simulink model "Single_Phase_HERIC_Inverter"  (R2023b)
settings: Solver=VariableStepAuto  StartTime=0.0  StopTime=0.5  RelTol=1e-3
libraries: spsSeriesRLCBranchLib x5, spsVoltageMeasurementLib x4, spsCurrentMeasurementLib x2, spsIGBTDiodeLib x2, spsMeanLib x2, spsACVoltageSourceLib x1, spsDCVoltageSourceLib x1, spsUniversalBridgeLib x1, powerlib_extras x1, spsRMSLib x1, spsTHDLib x1, spspowerguiLib x1
settings Model: SimulationMode=accelerator  Creator=abc6820292  LastModifiedBy=Qu
settings DataIOCC: ReturnWorkspaceOutputs=off
settings DebuggingCC: UnconnectedInputMsg=warning  UnconnectedOutputMsg=warning  UnconnectedLineMsg=warning
settings ModelReferenceCC: EnableRefExpFcnMdlSchedulingChecks=on
settings RTWCC: DLArmComputeVersion=19.05

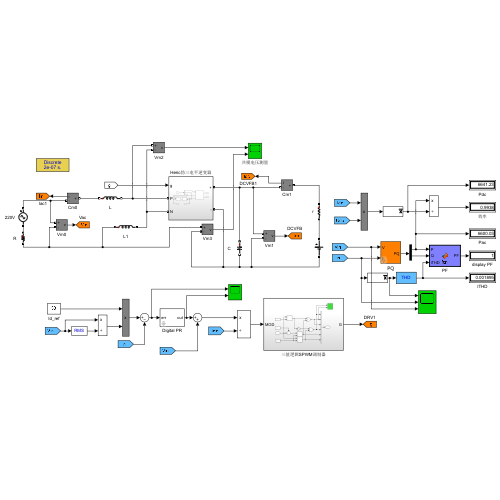
[thumbnail: Simulink's stored preview of the top-level diagram]
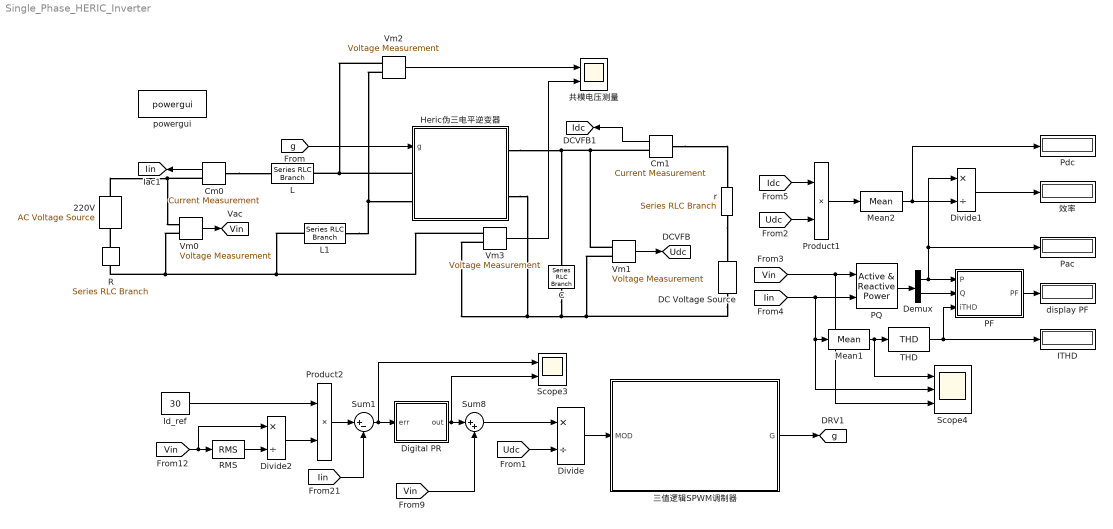
== system Single_Phase_HERIC_Inverter ==
  220V : spsACVoltageSourceLib/AC Voltage Source  Amplitude=220*1.414  Phase=0  Frequency=50  SampleTime=0  Measurements=None  BusType=swing  Pref=10e3  Qref=0  Qmin=-inf  Qmax=+inf
  C : spsSeriesRLCBranchLib/Series RLC Branch  LConnTagsString=__new0  RConnTagsString=__new0  BranchType=C  Resistance=0.01  Inductance=7e-4  SetiL0=off  InitialCurrent=0  Capacitance=2e-3  Setx0=on  InitialVoltage=360  Measurements=None
  Cm0 : spsCurrentMeasurementLib/Current Measurement  PhasorSimulation=off  OutputType=Complex  PSBequivalent=0
  Cm1 : spsCurrentMeasurementLib/Current Measurement  PhasorSimulation=off  OutputType=Complex  PSBequivalent=0
  DC Voltage Source : spsDCVoltageSourceLib/DC Voltage Source  Amplitude=360  Measurements=None
  Demux : Demux  Outputs=2
  Digital PR : Subsystem  mask{Kp=6, Kr=100, Wc=5, Ts=1/40000, Upper=400, Lower=-400}
      mask DialogControl ParameterGroupVar Prompt: 参数
  Divide : Product  Inputs=*/
  Divide1 : Product  Inputs=*/
  Divide2 : Product  Inputs=*/
  Heric伪三电平逆变器 : Subsystem
  ITHD : Display
  Id_ref : Constant  Value=30
  L : spsSeriesRLCBranchLib/Series RLC Branch  LConnTagsString=__new0  RConnTagsString=__new0  BranchType=L  Resistance=0.05  Inductance=3e-4  SetiL0=off  InitialCurrent=0  Capacitance=1e-3  Setx0=off  InitialVoltage=0  Measurements=None
  L1 : spsSeriesRLCBranchLib/Series RLC Branch  LConnTagsString=__new0  RConnTagsString=__new0  BranchType=L  Resistance=0.05  Inductance=3e-4  SetiL0=off  InitialCurrent=0  Capacitance=1e-3  Setx0=off  InitialVoltage=0  Measurements=None
  Mean1 : spsMeanLib/Mean  Freq=10000  Vinit=0  Ts=0
  Mean2 : spsMeanLib/Mean  Freq=50  Vinit=0  Ts=0
  PF : MATLAB Function  TreatAsAtomicUnit=on
  PQ : powerlib_extras/Measurements/Active & Reactive Power  f1=50
  Pac : Display
      settings: Format=bank
  Pdc : Display
      settings: Format=bank
  Product1 : Product  RndMeth=Zero
  Product2 : Product  RndMeth=Zero
  R : spsSeriesRLCBranchLib/Series RLC Branch  LConnTagsString=__new0  RConnTagsString=__new0  BranchType=R  Resistance=0.01  Inductance=7e-4  SetiL0=off  InitialCurrent=0  Capacitance=1e-8  Setx0=off  InitialVoltage=200  Measurements=None
  RMS : spsRMSLib/RMS  TrueRMS=off  Freq=50  RMSInit=220  Ts=0
  Scope3 : Scope  NumInputPorts=2
  Scope4 : Scope  NumInputPorts=3
  Sum1 : Sum  Inputs=|+-
  Sum8 : Sum  Inputs=|++
  THD : spsTHDLib/THD  Freq=50  Ts=0
  Vm{0..3} (4 alike) : spsVoltageMeasurementLib/Voltage Measurement  PhasorSimulation=off  OutputType=Complex  PSBequivalent=0
  display PF : Display
  powergui : spspowerguiLib/powergui  SimulationMode=Discrete  SampleTime=2e-7  frequency=60  Iterations=50  frequencyindice=0  Pbase=100e6  ErrMax=1e-4  UnitsV=kV  UnitsW=MW  buscounter=0  FunctionMessages=off  echomessages=off  EnableUseOfTLC=off  CurrentSourceSwitches=off  DisableSnubberDevices=off  DisableRonSwitches=off  DisableVfSwitches=off  DisplayEquations=off  AutomaticDiscreteSolvers=off  SolverType=Tustin/Backward Euler (TBE)  Interpol=off  ExternalGateDelay=off  methode=off  Ts=0  x0status=blocks  SPID=off  SwTol=0  HookPort=off  NonlinearTolerance=1e-4  nMaxIteration=100  ContinueOnMaxIteration=off  RestoreLinks=warning  ResistiveCurrentMeasurement=off  Frange=[0:2:500]  Ylog=off  Xlog=on  ShowGrid=off  save=off  variable=ZData  structure=QQQQQ  ZoomFFT=off  StartTime=0.5  cycles=15  DisplayStyle=1  fundamental=50  FreqAxis=off  MaxFrequency=1000  frequencyindicesteady=1  RmsSteady=1  display=off
  r : spsSeriesRLCBranchLib/Series RLC Branch  LConnTagsString=__new0  RConnTagsString=__new0  BranchType=R  Resistance=0.05  Inductance=1e-4  SetiL0=off  InitialCurrent=0  Capacitance=1e-3  Setx0=off  InitialVoltage=0  Measurements=None
  三值逻辑SPWM调制器 : Subsystem
  共模电压测量 : Scope  NumInputPorts=2
  效率 : Display
  tag scope: Idc=global, Iin=global, Udc=global, Vin=global, g=global
  wires:
  [g] -> Heric伪三电平逆变器/1(g)
  Vm0/1 -> [Vin]
  Demux/2 -> PF/2(Q)
  PF/1(PF) -> display PF/1
  PQ/1 -> Demux/1
  THD/1 -> ITHD/1, PF/3(iTHD)
  [Vin] -> Scope4/3, PQ/1
  Demux/1 -> Divide1/1, Pac/1, PF/1(P)
  Vm1/1 -> [Udc]
  三值逻辑SPWM调制器/1(G) -> [g]
  Cm0/1 -> [Iin]
  Divide/1 -> 三值逻辑SPWM调制器/1(MOD)
  [Udc] -> Divide/2
  [Iin] -> Sum1/2
  [Iin] -> Scope4/2, Mean1/1, PQ/2
  Sum8/1 -> Divide/1
  [Vin] -> Sum8/2
  [Vin] -> Divide2/1, RMS/1
  RMS/1 -> Divide2/2
  Divide2/1 -> Product2/2
  Id_ref/1 -> Product2/1
  Mean1/1 -> Scope4/1, THD/1
  Sum1/1 -> Digital PR/1(err), Scope3/1
  Product2/1 -> Sum1/1
  Vm2/1 -> 共模电压测量/1
  Vm3/1 -> 共模电压测量/2
  Digital PR/1(out) -> Scope3/2, Sum8/1
  Cm1/1 -> [Idc]
  [Udc] -> Product1/2
  [Idc] -> Product1/1
  Product1/1 -> Mean2/1
  Mean2/1 -> Pdc/1, Divide1/2
  Divide1/1 -> 效率/1
  connections:
  Vm1/LConn1 -- Heric伪三电平逆变器/RConn1 -- C/LConn1 -- Cm1/RConn1
  DC Voltage Source/LConn1 -- C/RConn1 -- Vm3/LConn2 -- Heric伪三电平逆变器/RConn2 -- Vm1/LConn2
  Cm0/RConn1 -- 220V/RConn1 -- Vm0/LConn1
  Vm2/LConn2 -- L1/RConn1 -- Heric伪三电平逆变器/LConn2
  Cm0/LConn1 -- L/LConn1
  r/RConn1 -- DC Voltage Source/RConn1
  L/RConn1 -- Heric伪三电平逆变器/LConn1 -- Vm2/LConn1
  R/LConn1 -- 220V/LConn1
  Vm0/LConn2 -- Vm3/LConn1 -- L1/LConn1 -- R/RConn1
  Cm1/LConn1 -- r/LConn1

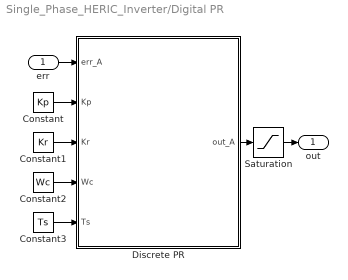
== system Single_Phase_HERIC_Inverter/Digital PR ==
  err : Inport
  Constant : Constant  Value=Kp
  Constant1 : Constant  Value=Kr
  Constant2 : Constant  Value=Wc
  Constant3 : Constant  Value=Ts
  Discrete PR : MATLAB Function  TreatAsAtomicUnit=on
  Saturation : Saturate  UpperLimit=Upper  LowerLimit=Lower
  out : Outport
  wires:
  Constant1/1 -> Discrete PR/3(Kr)
  Constant3/1 -> Discrete PR/5(Ts)
  Constant/1 -> Discrete PR/2(Kp)
  Constant2/1 -> Discrete PR/4(Wc)
  Discrete PR/1(out_A) -> Saturation/1
  Saturation/1 -> out/1
  err/1 -> Discrete PR/1(err_A)

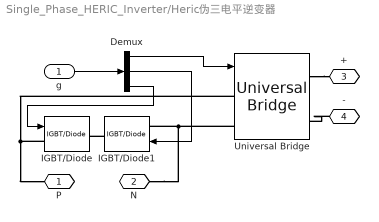
== system Single_Phase_HERIC_Inverter/Heric伪三电平逆变器 ==
  g : Inport
  Demux : Demux  Outputs=3
  IGBT/Diode : spsIGBTDiodeLib/IGBT//Diode  Ron=1e-3  Rs=1e5  Cs=inf  Measurements=off
  IGBT/Diode1 : spsIGBTDiodeLib/IGBT//Diode  Ron=1e-3  Rs=1e5  Cs=inf  Measurements=off
  Universal Bridge : spsUniversalBridgeLib/Universal Bridge  Arms=2  SnubberResistance=1e5  SnubberCapacitance=inf  Device=IGBT / Diodes  Ron=1e-3  Lon=0  ForwardVoltages="[  1  1  ]"  ForwardVoltage=0  GTOparameters=[ 10e-6 , 20e-6 ]  IGBTparameters=[ 1e-6 , 2e-6 ]  Measurements=None  Measurements_2=None  converterType=Rectifier
  P : PMIOPort  Side=Left
  N : PMIOPort  Port=2  Side=Left
  + : PMIOPort  Port=3  Side=Right
  - : PMIOPort  Port=4  Side=Right
  wires:
  g/1 -> Demux/1
  Demux/3 -> IGBT/Diode/1
  Demux/1 -> Universal Bridge/1
  Demux/2 -> IGBT/Diode1/1
  connections:
  IGBT/Diode1/RConn1 -- IGBT/Diode/RConn1
  IGBT/Diode/LConn1 -- Universal Bridge/LConn1 -- P/RConn1
  N/RConn1 -- Universal Bridge/LConn2 -- IGBT/Diode1/LConn1
  -/RConn1 -- Universal Bridge/RConn2
  Universal Bridge/RConn1 -- +/RConn1

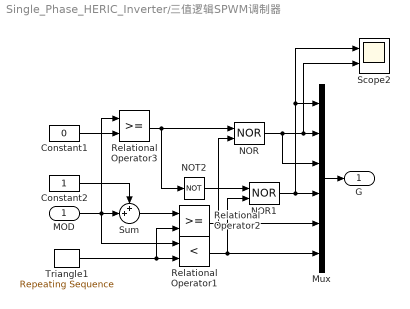
== system Single_Phase_HERIC_Inverter/三值逻辑SPWM调制器 ==
  MOD : Inport
  Constant1 : Constant  Value=0
  Constant2 : Constant
  Mux : Mux  Inputs=6
  NOR : Logic  Operator=NOR  IconShape=distinctive  AllPortsSameDT=off  OutDataTypeStr=boolean
  NOR1 : Logic  Operator=NOR  IconShape=distinctive  AllPortsSameDT=off  OutDataTypeStr=boolean
  NOT2 : Logic  Operator=NOT  IconShape=distinctive  AllPortsSameDT=off  OutDataTypeStr=boolean
  Relational Operator1 : RelationalOperator  Operator=<  OutDataTypeStr=boolean  InputSameDT=off
  Relational Operator2 : RelationalOperator  OutDataTypeStr=boolean  InputSameDT=off
  Relational Operator3 : RelationalOperator  OutDataTypeStr=boolean  InputSameDT=off
  Scope2 : Scope  NumInputPorts=2
  Sum : Sum  Inputs=++|
  Triangle1 : simulink/Sources/Repeating Sequence  rep_seq_t=[0 1/20000/2 1/20000]  rep_seq_y=[0 1 0]
  G : Outport
  wires:
  MOD/1 -> Relational Operator1/1, Relational Operator3/1, Sum/2
  Sum/1 -> Relational Operator2/1
  Mux/1 -> G/1
  Triangle1/1 -> Relational Operator2/2, Relational Operator1/2
  Constant2/1 -> Sum/1
  Constant1/1 -> Relational Operator3/2
  Relational Operator1/1 -> NOR1/2, Mux/6
  Relational Operator2/1 -> Mux/5, NOR/2
  Relational Operator3/1 -> NOT2/1, NOR/1
  NOR/1 -> Mux/3, Scope2/2, Mux/2
  NOR1/1 -> Scope2/1, Mux/1, Mux/4
  NOT2/1 -> NOR1/1

== matlab function Single_Phase_HERIC_Inverter/PF ==
  data: P input; PF output; Q input; iTHD input
function PF = fcn(P,Q,iTHD)
% This block supports an embeddable subset of the MATLAB language.
% See the help menu for details. 
PF=(P/sqrt(P*P+Q*Q))/(sqrt(1+iTHD*iTHD));

== matlab function Single_Phase_HERIC_Inverter/Digital PR/Discrete PR ==
  settings: updateMethod=DISCRETE  sampleTime=Ts
  data: err_A input; out_A output; Kp input; Kr input; Wc input; Ts input
function out_A  = fcn(err_A, Kp, Kr, Wc, Ts)

W0 = 50*2*pi;


persistent err_A1;
persistent err_A2;
persistent out_A1;
persistent out_A2;


%%对三相静态变量初始化
if isempty(err_A1)
    err_A1 = 0;
end
if isempty(err_A2)
    err_A2 = 0;
end
if isempty(out_A1)
    out_A1 = 0;
end
if isempty(out_A2)
    out_A2 = 0;
end


%%Discrete
t1 = Wc * Ts;
t2 = W0^2 * Ts^2;
t3 = t2 + 4*t1 + 4;

b0 = (Kp*t2 + 4*(Kp+Kr)*t1 + 4*Kp) / t3;
b1 = (2*Kp*t2 - 8*Kp) / t3;
b2 = (Kp*t2 + 4*Kp - 4*(Kp+Kr)*t1) / t3;
a1 = (2*t2 - 8) / t3;
a2 = (t2 - 4*t1 + 4) / t3;
%%限制输出
if b0>3000
    b0=0;
end
if b0<-3000
    b0=0;
end

%%计算输出量
out_A = b0*err_A + b1*err_A1 + b2*err_A2 - a1*out_A1 - a2*out_A2;
out_A2 = out_A1;
out_A1 = out_A;
err_A2 = err_A1;
err_A1 = err_A;
